simulink library "Linkage"  (R2025b)
settings: Solver=VariableStepAuto  StartTime=0.0  StopTime=10.0  RelTol=1e-3
undefined symbols (not defined in the file): Axle1D, AxleIn, Chassis, Init, RaceFix, RaceSpin, Vehicle, Visual, X, Y, Z
libraries: sm_lib x940, nesl_utility x136, fl_lib x6, Linkage_Systems x2, SteeringWheel x2, Linkage_Decoupled x2, AntiRollBar_Systems x1, Steer_Rack_None x1, Steer_Rack_WheelDrivenRack1UJoint x1
(part 1 of 25)
settings Model: Creator=andrei  LastModifiedBy=andrei

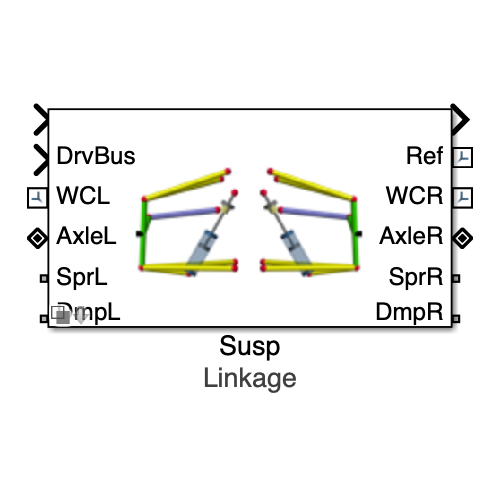
[thumbnail: Simulink's stored preview of the top-level diagram]
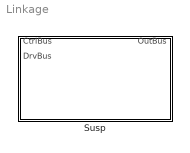
== system Linkage ==
  Susp : Subsystem  Variant=on  VariantControlMode=label  VariantControl=Variant1  LabelModeActiveChoice=Linkage  mask(Suspension and Steering){Susp=Chassis.SuspA1, Init=Init.Axle1, VariantLabel=Chassis.SuspA1.class.Value}
      mask prompts: Susp "Suspension Parameters"; Init "Initial Values"; VariantLabel "Variant Label"
      mask help: Models suspension and optional steering system for one axle. Option is chosen by string provided in Variant Label. The parameters for the selected option are contained in Suspension Parameters data structure.
      mask init:
      | curblk = gcb;
      | 
      | % Set variant for this block 
      | set_param(curblk,'LabelModeActiveChoice',VariantLabel);
      settings: AttributesFormatString=%<LabelModeActiveChoice>

== system Linkage/Susp ==
  "CtrlBus " : Inport
  DrvBus : Inport  Port=2
  Linkage : Subsystem  VariantControl=Linkage  mask(Linkage Suspension){}
      mask help: Models suspension using linkages, including double-wishbone and multi-link suspensions. This subsystem models the suspension, spring and damper parts, and optional steering system. The displacement of the springs and dampers are modeled here and the forces are modeled in a separate subsystem.
      mask Display: image('sm_car_vehicle_susp_linkage_IMAGE.png');
  Linkage Decoupled : Subsystem  VariantControl=Decoupled  mask(Linkage Decoupled){}
      mask help: Models suspension using a linkage where the stiffness and damping for the roll and heave degrees of freedom are decoupled. Includes suspension, spring and damper parts, and optional steering system. The displacement of the springs and dampers are modeled here and the forces are modeled in a separate subsystem.
      mask Display: image('sm_car_vehicle_susp_linkage_decouple_IMAGE.png');
  WCL : PMIOPort  Side=Left
  Ref : PMIOPort  Port=2  Side=Right
  WCR : PMIOPort  Port=3  Side=Right
  AxleL : PMIOPort  Port=4  Side=Left
  AxleR : PMIOPort  Port=5  Side=Right
  SprL : PMIOPort  Port=6  Side=Left
  SprR : PMIOPort  Port=7  Side=Right
  DmpL : PMIOPort  Port=8  Side=Left
  DmpR : PMIOPort  Port=9  Side=Right
  OutBus : Outport  VectorParamsAs1DForOutWhenUnconnected=off

== system Linkage/Susp/Linkage ==
  In Bus Element : Inport  PortName=CtrlBus  Element=Steer
  DrvBus : Inport  Port=2
  Anti Roll Bar : AntiRollBar_Systems/Anti Roll Bar  LabelModeActiveChoice=DroplinkRod  AntiRollBar=Susp.AntiRollBar  VariantLabel=Susp.AntiRollBar.class.Value
      settings: AttributesFormatString=%<LabelModeActiveChoice>
  Linkage L : Linkage_Systems/Linkage  VariantControl=Variant1  LabelModeActiveChoice=DoubleWishbone Pushrod  popup_leftRight=Left  Linkage=Susp.Linkage  InitLinkage=Init  VariantLabel=Susp.Linkage.class.Value
      settings: AttributesFormatString=%<ActiveVariant>
  Linkage R : Linkage_Systems/Linkage  VariantControl=Variant1  LabelModeActiveChoice=DoubleWishbone Pushrod  popup_leftRight=Right  Linkage=Susp.Linkage  InitLinkage=Init  VariantLabel=Susp.Linkage.class.Value
      settings: AttributesFormatString=%<ActiveVariant>
  Simscape Bus L : SimscapeBus  HierarchyStrings=RaceSpin;RaceFix;Axle1D;AxleIn
  Simscape Bus L1 : SimscapeBus  HierarchyStrings=RaceSpin;RaceFix;Axle1D;AxleIn
  Steer : Subsystem  Variant=on  VariantControlMode=label  VariantControl=Steer  LabelModeActiveChoice=RackWheel  mask{Steer=Susp.Steer, VariantLabel=Susp.Steer.class.Value}
      mask prompts: Steer "Steer Parameters"; VariantLabel "Variant Label"
      mask init:
      | curblk = gcb;
      | 
      | % Set variant for this block 
      | set_param(curblk,'LabelModeActiveChoice',VariantLabel);
      settings: AttributesFormatString=%<ActiveVariant>
      mask Display: disp(' ');
  Wheel Meas Left : Subsystem  mask(Wheel Measurements){popup_leftRight=Left}
      mask prompts: popup_leftRight "Left/Right"
      mask help: Calculates toe and camber angles based on orientation of wheel spin axis. To estimate steering axis inclination, the same measurements are done along the longitudinal axis (X) of the tire. Set Left/Right so that the sign of the logged toe and camber angles is associated with towards/away from vehicle center.
      mask init:
      | if(popup_leftRight == 1)
      |     rhs_tc = 1;
      | elseif(popup_leftRight == 2)
      |     rhs_tc = -1;
      | end
      mask TypeOptions popup_leftRight: Left | Right
  Wheel Meas Right : Subsystem  mask(Wheel Measurements){popup_leftRight=Right}
      mask prompts: popup_leftRight "Left/Right"
      mask help: Calculates toe and camber angles based on orientation of wheel spin axis. To estimate steering axis inclination, the same measurements are done along the longitudinal axis (X) of the tire. Set Left/Right so that the sign of the logged toe and camber angles is associated with towards/away from vehicle center.
      mask init:
      | if(popup_leftRight == 1)
      |     rhs_tc = 1;
      | elseif(popup_leftRight == 2)
      |     rhs_tc = -1;
      | end
      mask TypeOptions popup_leftRight: Left | Right
  WCL : PMIOPort  Side=Left
  Ref : PMIOPort  Port=2  Side=Right
  WCR : PMIOPort  Port=3  Side=Right
  AxleL : PMIOPort  Port=4  Side=Left
  AxleR : PMIOPort  Port=5  Side=Right
  SprL : PMIOPort  Port=6  Side=Left
  SprR : PMIOPort  Port=7  Side=Right
  DmpL : PMIOPort  Port=8  Side=Left
  DmpR : PMIOPort  Port=9  Side=Right
  Out Bus Element : Outport  VectorParamsAs1DForOutWhenUnconnected=off  PortName=OutBus  Element=Steer
  Out Bus Element1 : Outport  VectorParamsAs1DForOutWhenUnconnected=off  PortName=OutBus  Element=AntiRollBar
  Out Bus Element2 : Outport  VectorParamsAs1DForOutWhenUnconnected=off  PortName=OutBus  Element=WhlL
  Out Bus Element3 : Outport  VectorParamsAs1DForOutWhenUnconnected=off  PortName=OutBus  Element=WhlR
  Out Bus Element4 : Outport  VectorParamsAs1DForOutWhenUnconnected=off  PortName=OutBus  Element=LinkageR
  Out Bus Element5 : Outport  VectorParamsAs1DForOutWhenUnconnected=off  PortName=OutBus  Element=LinkageL
  wires:
  Wheel Meas Right/1(meas) -> Out Bus Element3/1
  Wheel Meas Left/1(meas) -> Out Bus Element2/1
  Anti Roll Bar/1 -> Out Bus Element1/1
  In Bus Element/1 -> Steer/2(CtrlBus)
  Steer/1(" meas") -> Out Bus Element/1
  DrvBus/1 -> Steer/1(DrvBus)
  Linkage R/1 -> Out Bus Element4/1
  Linkage L/1 -> Out Bus Element5/1
  connections:
  Linkage L/LConn8 -- Anti Roll Bar/LConn1
  Linkage R/LConn8 -- Anti Roll Bar/LConn3
  Linkage R/LConn5 -- Simscape Bus L1/LConn4
  Linkage L/LConn6 -- SprL/RConn1
  Simscape Bus L1/RConn1 -- AxleR/RConn1
  Linkage R/LConn4 -- Simscape Bus L1/LConn3
  Linkage R/LConn3 -- Simscape Bus L1/LConn2
  Linkage R/LConn2 -- Simscape Bus L1/LConn1
  Linkage R/LConn6 -- SprR/RConn1
  Linkage R/LConn7 -- DmpR/RConn1
  AxleL/RConn1 -- Simscape Bus L/RConn1
  Linkage L/LConn4 -- Simscape Bus L/LConn3
  Linkage L/LConn3 -- Simscape Bus L/LConn2
  Linkage L/LConn2 -- Simscape Bus L/LConn1
  Linkage L/LConn5 -- Simscape Bus L/LConn4
  Linkage L/LConn7 -- DmpL/RConn1
  Linkage L/RConn1 -- Steer/RConn1
  Wheel Meas Right/LConn2 -- Linkage R/LConn1 -- WCR/RConn1
  Wheel Meas Left/LConn2 -- Linkage L/LConn1 -- WCL/RConn1
  Wheel Meas Left/LConn1 -- Wheel Meas Right/LConn1 -- Steer/RConn2 -- Linkage R/RConn2 -- Linkage L/RConn2 -- Anti Roll Bar/LConn2 -- Ref/RConn1
  Linkage R/RConn1 -- Steer/RConn3

== system Linkage/Susp/Linkage Decoupled ==
  In Bus Element : Inport  PortName=CtrlBus  Element=Steer
  DrvBus : Inport  Port=2
  Linkage L : Linkage_Decoupled/Linkage  VariantControl=Variant1  LabelModeActiveChoice=DWDecoupled  popup_leftRight=Left  Linkage=Susp.Linkage  InitLinkage=Init  VariantLabel=Susp.Linkage.class.Value
      settings: AttributesFormatString=%<ActiveVariant>
  Linkage R : Linkage_Decoupled/Linkage  VariantControl=Variant1  LabelModeActiveChoice=DWDecoupled  popup_leftRight=Right  Linkage=Susp.Linkage  InitLinkage=Init  VariantLabel=Susp.Linkage.class.Value
      settings: AttributesFormatString=%<ActiveVariant>
  RollHeave Decouple : Subsystem  VariantControl=Variant1  mask(Roll and Heave Spring Dampers){hp_pushrod=Susp.Linkage.Pushrod.sBellcrank.Value, hp_bcr_pivot=Susp.Linkage.Bellcrank.sPivot.Value, hp_bcr_shock_heaveL=Susp.Linkage.Shock.Heave.sLeft.Value, hp_bcr_shock_heaveR=Susp.Linkage.Shock.Heave.sRight.Value, hp_bcr_shock_rollL=Susp.Linkage.Shock.Roll.sLeft.Value, hp_bcr_shock_rollR=Susp.Linkage.Shock.Roll.sRight.Value, shock_pist_mass_heave=Susp.Linkage.Shock.Heave.mPiston.Value, shock_pist_mass_roll=Susp.Linkage.Shock.Roll.mPiston.Value, shock_cyl_mass_heave=Susp.Linkage.Shock.Heave.mCylinder.Value, shock_cyl_mass_roll=Susp.Linkage.Shock.Roll.mCylinder.Value, up_lim_bumpstop_heave=Susp.Linkage.Endstop.Heave.xMax.Value, up_lim_bumpstop_roll=Susp.Linkage.Endstop.Roll.xMax.Value, low_lim_bumpstop_heave=Susp.Linkage.Endstop.Heave.xMin.Value, low_lim_bumpstop_roll=Susp.Linkage.Endstop.Roll.xMin.Value, clr_conn_shock=Visual.hp.clr, opc_conn_shock=Visual.hp.opc, size_conn_shock=Visual.hp.rad, clr_shock_cyl=Visual.Shock.cyl.clr, opc_shock_cyl=Visual.part.opc, radius_shock_cyl=Visual.Shock.cyl.rad, clr_shock_piston=Visual.Shock.piston.clr, opc_shock_piston=Visual.part.opc, clr_shock_bumpstop=Visual.Shock.bumpstop.clr, opc_shock_bumpstop=Visual.part.opc, deadvol_len_shock_cyl=Visual.Shock.dead_length, piston_len_shock=Visual.Shock.piston.len, cyl_cap_len_shock=Visual.Shock.cap.len, bumpstop_len_shock=Visual.Shock.bumpstop.len}
      mask prompts: hp_pushrod "HP Pushrod Inner  [xyz] (m)"; hp_bcr_pivot "HP Bellcrank Pivot [xyz] (m)"; deadvol_len_shock_cyl "Dead Volume Height (m)"; piston_len_shock "Piston Length (m)"; cyl_cap_len_shock "Cylinder Cap Length (m)"; bumpstop_len_shock "Bumpstop Length (m)"
      mask help: Models springs and dampers in a suspension design that decouples stiffness and damping for body roll and heave.
      mask init:
      | % Code to mirror hardpoint about vehicle xz plane
      | % and the plane defined by the bellcrank pivot axis
      | % and the y axis of the vehicle
      | % Code not used so that points can be specified independently
      | % Left here as a reference.
      | %{
      |  
      | a1 = atan2(hp_pushrod(1)-hp_bcr_pivot(1)   ,hp_pushrod(3)-hp_bcr_pivot(3));
      | a2 = atan2(hp_bcr_shock_roll(1)-hp_bcr_pivot(1),hp_bcr_shock_roll(3)-hp_bcr_pivot(3));
      | d_roll2piv = norm(hp_bcr_shock_roll([1 3])-hp_bcr_pivot([1 3]));
      | d_roll_mirror_axis = d_roll2piv*cos(a2-a1);
      | mirr_dx = d_roll_mirror_axis*sin(a1);
      | mirr_dz = d_roll_mirror_axis*cos(a1);
      | hp_bcr_shock_roll_r = ...
      |     [hp_bcr_shock_roll(1)-2*mirr_dx -hp_bcr_shock_roll(2) hp_bcr_shock_roll(3)-2*mirr_dz]
      | %}
      mask TypeOptions shock_pist_mass_heave: Shock Heave/shock_pist_mass
      mask TypeOptions shock_pist_mass_roll: Shock Roll/shock_pist_mass
      mask TypeOptions shock_cyl_mass_heave: Shock Heave/shock_cyl_mass
      mask TypeOptions shock_cyl_mass_roll: Shock Roll/shock_cyl_mass
      mask TypeOptions up_lim_bumpstop_heave: Shock Heave/up_lim_bumpstop
      mask TypeOptions up_lim_bumpstop_roll: Shock Roll/up_lim_bumpstop
      mask TypeOptions low_lim_bumpstop_heave: Shock Heave/low_lim_bumpstop
      mask TypeOptions low_lim_bumpstop_roll: Shock Roll/low_lim_bumpstop
      mask TypeOptions clr_conn_shock: Shock Heave/clr_conn_shock | Shock Roll/clr_conn_shock
      mask TypeOptions opc_conn_shock: Shock Heave/opc_conn_shock | Shock Roll/opc_conn_shock
      mask TypeOptions size_conn_shock: Shock Heave/size_conn_shock | Shock Roll/size_conn_shock
      mask TypeOptions clr_shock_cyl: Shock Heave/clr_shock_cyl | Shock Roll/clr_shock_cyl
      mask TypeOptions opc_shock_cyl: Shock Heave/opc_shock_cyl | Shock Roll/opc_shock_cyl
      mask TypeOptions radius_shock_cyl: Shock Heave/radius_shock_cyl | Shock Roll/radius_shock_cyl
      mask TypeOptions clr_shock_piston: Shock Heave/clr_shock_piston | Shock Roll/clr_shock_piston
      mask TypeOptions opc_shock_piston: Shock Heave/opc_shock_piston | Shock Roll/opc_shock_piston
      mask TypeOptions clr_shock_bumpstop: Shock Heave/clr_shock_bumpstop | Shock Roll/clr_shock_bumpstop
      mask TypeOptions opc_shock_bumpstop: Shock Heave/opc_shock_bumpstop | Shock Roll/opc_shock_bumpstop
      mask TypeOptions deadvol_len_shock_cyl: Shock Heave/deadvol_len_shock_cyl | Shock Roll/deadvol_len_shock_cyl
      mask TypeOptions piston_len_shock: Shock Heave/piston_len_shock | Shock Roll/piston_len_shock
      mask TypeOptions cyl_cap_len_shock: Shock Heave/cyl_cap_len_shock | Shock Roll/cyl_cap_len_shock
      mask TypeOptions bumpstop_len_shock: Shock Heave/bumpstop_len_shock | Shock Roll/bumpstop_len_shock
      mask DialogControl cont_hp Prompt: Hardpoints
      mask DialogControl text_hp_left Prompt: Left
      mask DialogControl text_hp_right Prompt: Right
      mask DialogControl text_hp_heave Prompt: Heave [xyz] (m)
      mask DialogControl text_hp_roll Prompt: Roll [xyz] (m)
      mask DialogControl cont_shock Prompt: Shock
      mask DialogControl text_shock_parts_blank Prompt: Parts
      mask DialogControl text_shock_heave Prompt: Heave
      mask DialogControl text_shock_roll Prompt: Roll
      mask DialogControl text_shock_pistm Prompt: Piston Mass (kg)
      mask DialogControl text_shock_cylm Prompt: Cylinder Mass (kg)
      mask DialogControl text_shock_bumpstop_par Prompt: Bumpstop
      mask DialogControl text_bump_ul Prompt: Upper Limit (m)
      mask DialogControl text_bump_low Prompt: Lower Limit (m)
      mask DialogControl cont_vis_shock Prompt: Visualization
      mask DialogControl text_clr_shock Prompt: Color  [RGB]
      mask DialogControl text_opc_shock Prompt: Opac. (0-1)
      mask DialogControl text_size_shock Prompt: Size (m)
      mask DialogControl text_conn_shock Prompt: Connections
      mask DialogControl text_shock_shock Prompt: Cylinder
      mask DialogControl text_shock_piston Prompt: Piston
      mask DialogControl text_piston_radius Prompt: <cylinder radius>
      mask DialogControl text_shock_bumpstop Prompt: Bumpstop
      mask DialogControl text_bumpstop_radius Prompt: <cylinder radius>
      mask Display: image('sm_car_vehicle_linkage_rollHeaveDecouple_IMAGE.png');
  Simscape Bus L : SimscapeBus  HierarchyStrings=RaceSpin;RaceFix;Axle1D;AxleIn
  Simscape Bus L1 : SimscapeBus  HierarchyStrings=RaceSpin;RaceFix;Axle1D;AxleIn
  Steer : Subsystem  Variant=on  VariantControlMode=label  VariantControl=Steer  LabelModeActiveChoice=WheelDrivenRack1UJoint  mask{Steer=Susp.Steer, VariantLabel=Susp.Steer.class.Value}
      mask prompts: Steer "Steer Parameters"; VariantLabel "Variant Label"
      mask init:
      | curblk = gcb;
      | 
      | % Set variant for this block 
      | set_param(curblk,'LabelModeActiveChoice',VariantLabel);
      settings: AttributesFormatString=%<ActiveVariant>
      mask Display: disp(' ');
  Wheel Meas Left : Subsystem  mask(Wheel Measurements){popup_leftRight=Left}
      mask prompts: popup_leftRight "Left/Right"
      mask help: Calculates toe and camber angles based on orientation of wheel spin axis. To estimate steering axis inclination, the same measurements are done along the longitudinal axis (X) of the tire. Set Left/Right so that the sign of the logged toe and camber angles is associated with towards/away from vehicle center.
      mask init:
      | if(popup_leftRight == 1)
      |     rhs_tc = 1;
      | elseif(popup_leftRight == 2)
      |     rhs_tc = -1;
      | end
      mask TypeOptions popup_leftRight: Left | Right
  Wheel Meas Right : Subsystem  mask(Wheel Measurements){popup_leftRight=Right}
      mask prompts: popup_leftRight "Left/Right"
      mask help: Calculates toe and camber angles based on orientation of wheel spin axis. To estimate steering axis inclination, the same measurements are done along the longitudinal axis (X) of the tire. Set Left/Right so that the sign of the logged toe and camber angles is associated with towards/away from vehicle center.
      mask init:
      | if(popup_leftRight == 1)
      |     rhs_tc = 1;
      | elseif(popup_leftRight == 2)
      |     rhs_tc = -1;
      | end
      mask TypeOptions popup_leftRight: Left | Right
  WCL : PMIOPort  Side=Left
  Ref : PMIOPort  Port=2  Side=Right
  WCR : PMIOPort  Port=3  Side=Right
  AxleL : PMIOPort  Port=4  Side=Left
  AxleR : PMIOPort  Port=5  Side=Right
  SprL : PMIOPort  Port=6  Side=Left
  SprR : PMIOPort  Port=7  Side=Right
  DmpL : PMIOPort  Port=8  Side=Left
  DmpR : PMIOPort  Port=9  Side=Right
  Out Bus Element : Outport  VectorParamsAs1DForOutWhenUnconnected=off  PortName=OutBus  Element=Steer
  Out Bus Element1 : Outport  VectorParamsAs1DForOutWhenUnconnected=off  PortName=OutBus  Element=RollHeave
  Out Bus Element2 : Outport  VectorParamsAs1DForOutWhenUnconnected=off  PortName=OutBus  Element=WhlL
  Out Bus Element3 : Outport  VectorParamsAs1DForOutWhenUnconnected=off  PortName=OutBus  Element=WhlR
  Out Bus Element4 : Outport  VectorParamsAs1DForOutWhenUnconnected=off  PortName=OutBus  Element=LinkageR
  Out Bus Element5 : Outport  VectorParamsAs1DForOutWhenUnconnected=off  PortName=OutBus  Element=LinkageL
  wires:
  Wheel Meas Right/1(meas) -> Out Bus Element3/1
  Wheel Meas Left/1(meas) -> Out Bus Element2/1
  In Bus Element/1 -> Steer/2(CtrlBus)
  Steer/1(" meas") -> Out Bus Element/1
  DrvBus/1 -> Steer/1(DrvBus)
  RollHeave Decouple/1(meas) -> Out Bus Element1/1
  Linkage R/1 -> Out Bus Element4/1
  Linkage L/1 -> Out Bus Element5/1
  connections:
  RollHeave Decouple/LConn1 -- Linkage L/LConn6
  Linkage R/LConn5 -- Simscape Bus L1/LConn4
  Simscape Bus L1/RConn1 -- AxleR/RConn1
  Linkage R/LConn4 -- Simscape Bus L1/LConn3
  Linkage R/LConn3 -- Simscape Bus L1/LConn2
  Linkage R/LConn2 -- Simscape Bus L1/LConn1
  AxleL/RConn1 -- Simscape Bus L/RConn1
  Linkage L/LConn4 -- Simscape Bus L/LConn3
  Linkage L/LConn3 -- Simscape Bus L/LConn2
  Linkage L/LConn2 -- Simscape Bus L/LConn1
  Linkage L/LConn5 -- Simscape Bus L/LConn4
  Steer/RConn1 -- Linkage L/RConn1
  Wheel Meas Right/LConn2 -- Linkage R/LConn1 -- WCR/RConn1
  Wheel Meas Left/LConn2 -- Linkage L/LConn1 -- WCL/RConn1
  Steer/RConn2 -- Wheel Meas Right/LConn1 -- Wheel Meas Left/LConn1 -- Linkage R/RConn2 -- Ref/RConn1 -- Linkage L/RConn2
  Steer/RConn3 -- Linkage R/RConn1
  RollHeave Decouple/LConn2 -- Linkage L/LConn7
  RollHeave Decouple/LConn7 -- Linkage R/LConn7
  RollHeave Decouple/LConn8 -- Linkage R/LConn6
  DmpL/RConn1 -- RollHeave Decouple/LConn4
  SprL/RConn1 -- RollHeave Decouple/LConn3
  DmpR/RConn1 -- RollHeave Decouple/LConn6
  SprR/RConn1 -- RollHeave Decouple/LConn5

== system Linkage/Susp/Linkage/Steer ==
  DrvBus : Inport
  CtrlBus : Inport  Port=2
  None : Steer_Rack_None/None  SystemSampleTime=-1  VariantControl=None  VariantActivationTime=update diagram  EmptyChoice=off  PassThrough=off  PassThroughVariantControl=(default)  EmptyChoiceVariantControl=(default)  AllowFlexibleInterface=on  Latency=0  AutoFrameSizeCalculation=off
  Rack Wheel : Subsystem  Tag=PublishSubsystem  AncestorBlock=Steer_Rack_Wheel/Rack Wheel  VariantControl=RackWheel  mask(Steering System with Rack Actuation){hp_wheel=Vehicle.Chassis.SuspA1.Steer.Wheel.sMount.Value, wheel_axis_incl=Vehicle.Chassis.SuspA1.Steer.Wheel.aAxis.Value, hp_mt_rack=Vehicle.Chassis.SuspA1.Steer.Rack.sMount.Value, hp_out_rack=Vehicle.Chassis.SuspA1.Steer.Rack.sOutboard.Value, Wheel=Steer.Wheel, rack_mass=Vehicle.Chassis.SuspA1.Steer.Rack.m.Value, whl2rack_whlangle=Vehicle.Chassis.SuspA1.Steer.Ratio_Table.aWheel.Value, whl2rack_rackdisp=Vehicle.Chassis.SuspA1.Steer.Ratio_Table.xRack.Value, whl2rack_filter=1/Vehicle.Chassis.SuspA1.Steer.Rack.fActuatorCutoff.Value, clr_rack=Visual.SteeringRack.clr, opc_rack=Visual.part.opc, radius_rack=Visual.SteeringRack.rad, clr_connhp=Visual.hp.clr, opc_connhp=Visual.hp.opc, size_connhp=Visual.hp.rad, clr_wheel=Visual.SteeringWheel.clr, opc_wheel=Visual.part.opc, DriverHuman=Steer.DriverHuman}
      mask prompts: hp_wheel "HP Wheel [xyz] (m)"; wheel_axis_incl "Wheel Axis Angle (rad)"; hp_mt_rack "HP Rack Mount [xyz] (m)"; hp_out_rack "HP Track Rod Inboard [xyz] (m)"; whl2rack_whlangle "Wheel Angle (deg)"; whl2rack_rackdisp "Rack Travel (m)"; whl2rack_filter "Rack Motion Filter (sec)"; DriverHuman "Driver Human (structure)"
      mask help: Steering wheel angle converted to rack displacement by lookup table. Steering wheel is present and rotates to match rack displacement (visualization only). Shafts are not present.
      mask TypeOptions hp_wheel:
      | Ref to Wheel/Transform
      | HP Wheel/TranslationCartesianOffset
      mask TypeOptions hp_mt_rack:
      | Ref to Rack/Transform
      | HP Rack/TranslationCartesianOffset
      mask TypeOptions hp_out_rack: Rack/hp_out
      mask TypeOptions rack_mass: Rack/rack_mass
      mask TypeOptions whl2rack_whlangle:
      | Wheel Angle to
      | Rack Displacement/BreakpointsForDimension1
      mask TypeOptions whl2rack_rackdisp:
      | Wheel Angle to
      | Rack Displacement/Table
      mask TypeOptions whl2rack_filter: Physical Signal/InputFilterTimeConstant
      mask TypeOptions clr_rack: Rack/clr_rack
      mask TypeOptions opc_rack: Rack/opc_rack
      mask TypeOptions radius_rack: Rack/radius_rack
      mask TypeOptions clr_connhp:
      | Ref to Rack/Vis
      | Rack
      | Housing/GraphicDiffuseColor
      mask TypeOptions opc_connhp:
      | Ref to Rack/Vis
      | Rack
      | Housing/GraphicOpacity
      mask TypeOptions size_connhp:
      | Ref to Rack/Vis
      | Rack
      | Housing/SphereRadius
      mask TypeOptions clr_wheel: Wheel/clr_wheel
      mask TypeOptions opc_wheel: Wheel/opc_wheel
      mask DialogControl cont_steer Prompt: Steer
      mask DialogControl grp_strparts Prompt: Parts
      mask DialogControl text_strparts_len Prompt: Length/Radius (m)
      mask DialogControl text_strparts_mass Prompt: Mass (kg)
      mask DialogControl text_strparts_wheel Prompt: Wheel
      mask DialogControl text_strparts_wheel_m Prompt: <CAD file>
      mask DialogControl text_strparts_rack Prompt: Rack
      mask DialogControl text_strparts_rack_len Prompt: <HP Rod Inboard>
      mask DialogControl grp_whl2rack Prompt: Wheel to Rack
      mask DialogControl cont_vis_steer Prompt: Visualization
      mask DialogControl text_steer_vis_clr Prompt: Color [RGB]
      mask DialogControl text_steer_vis_opc Prompt: Opac. (0-1)
      mask DialogControl text_steer_vis_size Prompt: Size (m)
      mask DialogControl text_steer_vis_rack Prompt: Rack
      mask DialogControl text_steer_vis_connhp Prompt: Connections, HP
      mask DialogControl text_steer_vis_wheel Prompt: Wheel
      mask DialogControl text_wheel_size Prompt: <CAD File>
      mask DialogControl cont_driver_human Prompt: Driver Human
  Wheel Driven Rack 1UJoint : Steer_Rack_WheelDrivenRack1UJoint/Wheel Driven Rack 1UJoint  Tag=PublishSubsystem  VariantControl=WheelDrivenRack1UJoint  hp_wheel=Vehicle.Chassis.SuspA1.Steer.Wheel.sMount.Value  wheel_axis_incl=Vehicle.Chassis.SuspA1.Steer.Wheel.aAxis.Value  hp_mt_rack=Vehicle.Chassis.SuspA1.Steer.Rack.sMount.Value  hp_out_rack=Vehicle.Chassis.SuspA1.Steer.Rack.sOutboard.Value  hp_pinion=Vehicle.Chassis.SuspA1.Steer.Pinion.sMount.Value  Wheel=Steer.Wheel  len_sha_u=Vehicle.Chassis.SuspA1.Steer.Shaft_Upper.xLength.Value  sha_u_mass=Steer.Shaft_Upper.m.Value  sha_l_mass=Steer.Shaft_Lower.m.Value  rad_pinion=Vehicle.Chassis.SuspA1.Steer.Pinion.xRad.Value  pinion_mass=Steer.Pinion.m.Value  rack_mass=Steer.Rack.m.Value  whl2steer_filter=1/Vehicle.Chassis.SuspA1.Steer.Rack.fActuatorCutoff.Value  clr_rack=Visual.SteeringRack.clr  opc_rack=Visual.part.opc  radius_rack=Visual.SteeringRack.rad  clr_shaft=Visual.SteeringShafts.clr  opc_shaft=Visual.part.opc  size_shaft=Visual.SteeringShafts.rad  clr_pinion=Visual.SteeringPinion.clr  opc_pinion=Visual.part.opc  len_pinion=Visual.SteeringPinion.len  clr_connhp=Visual.hp.clr  opc_connhp=Visual.hp.opc  size_connhp=Visual.hp.rad  clr_wheel=Visual.SteeringWheel.clr  opc_wheel=Visual.part.opc  DriverHuman=Steer.DriverHuman
  Wheel Driven Rack 1UJoint1 : Subsystem  Tag=PublishSubsystem  VariantControl=WheelDrivenRack1UJoint1  mask(Steering System with Wheel Actuation){hp_wheel=Steer.Wheel.sMount.Value, wheel_axis_incl=Steer.Wheel.aAxis.Value, hp_mt_rack=Steer.Rack.sMount.Value, hp_out_rack=Steer.Rack.sOutboard.Value, hp_pinion=Steer.Pinion.sMount.Value, Wheel=Steer.Wheel, len_sha_u=Steer.Shaft_Upper.xLength.Value, sha_u_mass=Steer.Shaft_Upper.m.Value, sha_l_mass=Steer.Shaft_Lower.m.Value, rad_pinion=Steer.Pinion.xRad.Value, pinion_mass=Steer.Pinion.m.Value, rack_mass=Steer.Rack.m.Value, whl2steer_filter=1/Steer.Rack.fActuatorCutoff.Value, clr_rack=Visual.SteeringRack.clr, opc_rack=Visual.part.opc, radius_rack=Visual.SteeringRack.rad, clr_shaft=Visual.SteeringShafts.clr, opc_shaft=Visual.part.opc, size_shaft=Visual.SteeringShafts.rad, clr_pinion=Visual.SteeringPinion.clr, opc_pinion=Visual.part.opc, len_pinion=Visual.SteeringPinion.len, clr_connhp=Visual.hp.clr, opc_connhp=Visual.hp.opc, size_connhp=Visual.hp.rad, clr_wheel=Visual.SteeringWheel.clr, opc_wheel=Visual.part.opc, DriverHuman=Steer.DriverHuman}
      mask prompts: hp_wheel "HP Wheel [xyz] (m)"; wheel_axis_incl "Wheel Axis Angle (rad)"; hp_mt_rack "HP Rack Mount [xyz] (m)"; hp_out_rack "HP Track Rod Inboard [xyz] (m)"; hp_pinion "HP Pinion [xyz] (m)"; whl2steer_filter "Steer Motion Filter (sec)"; DriverHuman "Driver Human (structure)"
      mask help: Actuation is applied to steering wheel and transmitted to rack via shafts in steering column. Assumes constant gear ratio between pinion and rack.
      mask init:
      | % Calculate inclination of pinion gear about rack travel axis
      | pinion_incl = atan2(hp_mt_rack(1)-hp_pinion(1),hp_mt_rack(3)-hp_pinion(3));
      | 
      | % Calculate location of universal joint
      | hp_col_upper = hp_wheel  + [+len_sha_u*cos(wheel_axis_incl)  0 -len_sha_u*sin(wheel_axis_incl)];
      mask TypeOptions hp_wheel:
      | Ref to Wheel/Transform
      | HP Wheel/TranslationCartesianOffset
      mask TypeOptions hp_mt_rack:
      | Ref to Rack/Transform
      | HP Rack/TranslationCartesianOffset
      mask TypeOptions hp_out_rack: Rack/hp_out
      mask TypeOptions rack_mass: Rack/rack_mass
      mask TypeOptions whl2steer_filter: Physical Signal/InputFilterTimeConstant
      mask TypeOptions clr_rack: Rack/clr_rack
      mask TypeOptions opc_rack: Rack/opc_rack
      mask TypeOptions radius_rack: Rack/radius_rack
      mask TypeOptions clr_shaft:
      | Shaft
      | Steering/Shaft/GraphicDiffuseColor | Shaft
      | Lower/Shaft/GraphicDiffuseColor | Shaft
      | Intermediate/Shaft/GraphicDiffuseColor
      mask TypeOptions opc_shaft:
      | Shaft
      | Steering/Shaft/GraphicOpacity | Shaft
      | Lower/Shaft/GraphicOpacity | Shaft
      | Intermediate/Shaft/GraphicOpacity
      mask TypeOptions size_shaft:
      | Shaft
      | Steering/Shaft/CylinderRadius | Shaft
      | Lower/Shaft/CylinderRadius | Shaft
      | Intermediate/Shaft/CylinderRadius
      mask TypeOptions clr_pinion: Pinion/Pinion/GraphicDiffuseColor
      mask TypeOptions opc_pinion: Pinion/Pinion/GraphicOpacity
      mask TypeOptions len_pinion: Pinion/Pinion/CylinderLength
      mask TypeOptions clr_connhp:
      | Ref to Rack/Vis
      | Rack
      | Housing/GraphicDiffuseColor | HPs/HP Lower Col/GraphicDiffuseColor | HPs/HP Pinion/GraphicDiffuseColor | HPs/HP Upper Col/GraphicDiffuseColor
      mask TypeOptions opc_connhp:
      | Ref to Rack/Vis
      | Rack
      | Housing/GraphicOpacity | HPs/HP Lower Col/GraphicOpacity | HPs/HP Pinion/GraphicOpacity | HPs/HP Upper Col/GraphicOpacity
      mask TypeOptions size_connhp:
      | Ref to Rack/Vis
      | Rack
      | Housing/SphereRadius | HPs/HP Lower Col/SphereRadius | HPs/HP Pinion/SphereRadius | HPs/HP Upper Col/SphereRadius
      mask TypeOptions clr_wheel: Wheel/clr_wheel
      mask TypeOptions opc_wheel: Wheel/opc_wheel
      mask DialogControl cont_steer Prompt: Steer
      mask DialogControl grp_strparts Prompt: Parts
      mask DialogControl text_strparts_len Prompt: Length/Radius (m)
      mask DialogControl text_strparts_mass Prompt: Mass (kg)
      mask DialogControl text_strparts_wheel Prompt: Wheel
      mask DialogControl text_strparts_wheel_m Prompt: <CAD file>
      mask DialogControl text_strparts_sha_u Prompt: Upper Shaft
      mask DialogControl text_strparts_sha_i Prompt: Lower Shaft
      mask DialogControl text_strparts_sha_i_len Prompt: <length upper, lower>
      mask DialogControl text_strparts_pinion Prompt: Pinion
      mask DialogControl text_strparts_rack Prompt: Rack
      mask DialogControl text_strparts_rack_len Prompt: <HP Rod Inboard>
      mask DialogControl grp_steering Prompt: Steering Input
      mask DialogControl cont_vis_steer Prompt: Visualization
      mask DialogControl text_steer_vis_clr Prompt: Color [RGB]
      mask DialogControl text_steer_vis_opc Prompt: Opac. (0-1)
      mask DialogControl text_steer_vis_size Prompt: Size (m)
      mask DialogControl text_steer_vis_rack Prompt: Rack
      mask DialogControl text_steer_vis_shafts Prompt: Shafts
      mask DialogControl text_steer_vis_pinion Prompt: Pinion
      mask DialogControl text_steer_vis_connhp Prompt: Connections, HP
      mask DialogControl text_steer_vis_wheel Prompt: Wheel
      mask DialogControl text_steer_size_wheel Prompt: <CAD File>
      mask DialogControl cont_driver_human Prompt: Driver Human
  Wheel Driven Rack 1UJoint2 : Subsystem  Tag=PublishSubsystem  VariantControl=WheelDrivenRack1UJoint2  mask(Steering System with Wheel Actuation){hp_wheel=Steer.Wheel.sMount.Value, wheel_axis_incl=Steer.Wheel.aAxis.Value, hp_mt_rack=Steer.Rack.sMount.Value, hp_out_rack=Steer.Rack.sOutboard.Value, hp_pinion=Steer.Pinion.sMount.Value, Wheel=Steer.Wheel, len_sha_u=Steer.Shaft_Upper.xLength.Value, sha_u_mass=Steer.Shaft_Upper.m.Value, sha_l_mass=Steer.Shaft_Lower.m.Value, rad_pinion=Steer.Pinion.xRad.Value, pinion_mass=Steer.Pinion.m.Value, rack_mass=Steer.Rack.m.Value, whl2steer_filter=1/Steer.Rack.fActuatorCutoff.Value, clr_rack=Visual.SteeringRack.clr, opc_rack=Visual.part.opc, radius_rack=Visual.SteeringRack.rad, clr_shaft=Visual.SteeringShafts.clr, opc_shaft=Visual.part.opc, size_shaft=Visual.SteeringShafts.rad, clr_pinion=Visual.SteeringPinion.clr, opc_pinion=Visual.part.opc, len_pinion=Visual.SteeringPinion.len, clr_connhp=Visual.hp.clr, opc_connhp=Visual.hp.opc, size_connhp=Visual.hp.rad, clr_wheel=Visual.SteeringWheel.clr, opc_wheel=Visual.part.opc, DriverHuman=Steer.DriverHuman}
      mask prompts: hp_wheel "HP Wheel [xyz] (m)"; wheel_axis_incl "Wheel Axis Angle (rad)"; hp_mt_rack "HP Rack Mount [xyz] (m)"; hp_out_rack "HP Track Rod Inboard [xyz] (m)"; hp_pinion "HP Pinion [xyz] (m)"; whl2steer_filter "Steer Motion Filter (sec)"; DriverHuman "Driver Human (structure)"
      mask help: Actuation is applied to steering wheel and transmitted to rack via shafts in steering column. Assumes constant gear ratio between pinion and rack.
      mask init: same as Linkage/Susp/Linkage/Steer/Wheel Driven Rack 1UJoint1
      mask TypeOptions hp_wheel:
      | Ref to Wheel/Transform
      | HP Wheel/TranslationCartesianOffset
      mask TypeOptions hp_mt_rack:
      | Ref to Rack/Transform
      | HP Rack/TranslationCartesianOffset
      mask TypeOptions hp_out_rack: Rack/hp_out
      mask TypeOptions rack_mass: Rack/rack_mass
      mask TypeOptions whl2steer_filter: Physical Signal/InputFilterTimeConstant
      mask TypeOptions clr_rack: Rack/clr_rack
      mask TypeOptions opc_rack: Rack/opc_rack
      mask TypeOptions radius_rack: Rack/radius_rack
      mask TypeOptions clr_shaft:
      | Shaft
      | Steering/Shaft/GraphicDiffuseColor | Shaft
      | Lower/Shaft/GraphicDiffuseColor | Shaft
      | Intermediate/Shaft/GraphicDiffuseColor
      mask TypeOptions opc_shaft:
      | Shaft
      | Steering/Shaft/GraphicOpacity | Shaft
      | Lower/Shaft/GraphicOpacity | Shaft
      | Intermediate/Shaft/GraphicOpacity
      mask TypeOptions size_shaft:
      | Shaft
      | Steering/Shaft/CylinderRadius | Shaft
      | Lower/Shaft/CylinderRadius | Shaft
      | Intermediate/Shaft/CylinderRadius
      mask TypeOptions clr_pinion: Pinion/Pinion/GraphicDiffuseColor
      mask TypeOptions opc_pinion: Pinion/Pinion/GraphicOpacity
      mask TypeOptions len_pinion: Pinion/Pinion/CylinderLength
      mask TypeOptions clr_connhp:
      | Ref to Rack/Vis
      | Rack
      | Housing/GraphicDiffuseColor | HPs/HP Lower Col/GraphicDiffuseColor | HPs/HP Pinion/GraphicDiffuseColor | HPs/HP Upper Col/GraphicDiffuseColor
      mask TypeOptions opc_connhp:
      | Ref to Rack/Vis
      | Rack
      | Housing/GraphicOpacity | HPs/HP Lower Col/GraphicOpacity | HPs/HP Pinion/GraphicOpacity | HPs/HP Upper Col/GraphicOpacity
      mask TypeOptions size_connhp:
      | Ref to Rack/Vis
      | Rack
      | Housing/SphereRadius | HPs/HP Lower Col/SphereRadius | HPs/HP Pinion/SphereRadius | HPs/HP Upper Col/SphereRadius
      mask TypeOptions clr_wheel: Wheel/clr_wheel
      mask TypeOptions opc_wheel: Wheel/opc_wheel
      mask DialogControl cont_steer Prompt: Steer
      mask DialogControl grp_strparts Prompt: Parts
      mask DialogControl text_strparts_len Prompt: Length/Radius (m)
      mask DialogControl text_strparts_mass Prompt: Mass (kg)
      mask DialogControl text_strparts_wheel Prompt: Wheel
      mask DialogControl text_strparts_wheel_m Prompt: <CAD file>
      mask DialogControl text_strparts_sha_u Prompt: Upper Shaft
      mask DialogControl text_strparts_sha_i Prompt: Lower Shaft
      mask DialogControl text_strparts_sha_i_len Prompt: <length upper, lower>
      mask DialogControl text_strparts_pinion Prompt: Pinion
      mask DialogControl text_strparts_rack Prompt: Rack
      mask DialogControl text_strparts_rack_len Prompt: <HP Rod Inboard>
      mask DialogControl grp_steering Prompt: Steering Input
      mask DialogControl cont_vis_steer Prompt: Visualization
      mask DialogControl text_steer_vis_clr Prompt: Color [RGB]
      mask DialogControl text_steer_vis_opc Prompt: Opac. (0-1)
      mask DialogControl text_steer_vis_size Prompt: Size (m)
      mask DialogControl text_steer_vis_rack Prompt: Rack
      mask DialogControl text_steer_vis_shafts Prompt: Shafts
      mask DialogControl text_steer_vis_pinion Prompt: Pinion
      mask DialogControl text_steer_vis_connhp Prompt: Connections, HP
      mask DialogControl text_steer_vis_wheel Prompt: Wheel
      mask DialogControl text_steer_size_wheel Prompt: <CAD File>
      mask DialogControl cont_driver_human Prompt: Driver Human
  Wheel Driven Rack 1UJoint3 : Subsystem  Tag=PublishSubsystem  AncestorBlock=|  VariantControl=WheelDrivenRack1UJoint3  mask(Steering System with Wheel Actuation){hp_wheel=Steer.Wheel.sMount.Value, wheel_axis_incl=Steer.Wheel.aAxis.Value, hp_mt_rack=Steer.Rack.sMount.Value, hp_out_rack=Steer.Rack.sOutboard.Value, Wheel=Steer.Wheel, len_sha_u=Steer.Shaft_Upper.xLength.Value, sha_u_mass=Steer.Shaft_Upper.m.Value, sha_l_mass=Steer.Shaft_Lower.m.Value, rad_pinion=Steer.Pinion.xRad.Value, pinion_mass=Steer.Pinion.m.Value, rack_mass=Steer.Rack.m.Value, whl2steer_filter=1/Steer.Rack.fActuatorCutoff.Value, clr_rack=Visual.SteeringRack.clr, opc_rack=Visual.part.opc, radius_rack=Visual.SteeringRack.rad, clr_shaft=Visual.SteeringShafts.clr, opc_shaft=Visual.part.opc, size_shaft=Visual.SteeringShafts.rad, clr_pinion=Visual.SteeringPinion.clr, opc_pinion=Visual.part.opc, len_pinion=Visual.SteeringPinion.len, clr_connhp=Visual.hp.clr, opc_connhp=Visual.hp.opc, size_connhp=Visual.hp.rad, clr_wheel=Visual.SteeringWheel.clr, opc_wheel=Visual.part.opc, DriverHuman=Steer.DriverHuman}
      | Steer_Rack_WheelDrivenRack1UJoint/Wheel
      | Driven
      | Rack
      | 1UJoint
      mask prompts: hp_wheel "HP Wheel [xyz] (m)"; wheel_axis_incl "Wheel Axis Angle (rad)"; hp_mt_rack "HP Rack Mount [xyz] (m)"; hp_out_rack "HP Track Rod Inboard [xyz] (m)"; whl2steer_filter "Steer Motion Filter (sec)"; DriverHuman "Driver Human (structure)"
      mask help: Actuation is applied to steering wheel and transmitted to rack via shafts in steering column. Assumes constant gear ratio between pinion and rack.
      mask init:
      | % Calculate the pinion inclination only based on pinion radius, wheel and
      | % rack position
      | len = norm(hp_wheel - hp_mt_rack);
      | x1 = asin(rad_pinion/len);
      | x2 = atan2(abs(hp_wheel(1) - hp_mt_rack(1)),hp_wheel(3) - hp_mt_rack(3));
      | pinion_incl = pi/2 - x2 + x1;
      | 
      | % Calcule pinion hardpoint 
      | hp_pinion = hp_mt_rack - [cos(pinion_incl) * rad_pinion, 0, sin(pinion_incl) * rad_pinion];
      | 
      | % Calculate location of universal joint
      | hp_ujoint = hp_wheel  - (hp_wheel - hp_pinion)/2;
      mask TypeOptions hp_wheel:
      | Ref to Wheel/Transform
      | HP Wheel/TranslationCartesianOffset
      mask TypeOptions hp_mt_rack:
      | Ref to Rack/Transform
      | HP Rack/TranslationCartesianOffset
      mask TypeOptions hp_out_rack: Rack/hp_out
      mask TypeOptions rack_mass: Rack/rack_mass
      mask TypeOptions whl2steer_filter: Physical Signal/InputFilterTimeConstant
      mask TypeOptions clr_rack: Rack/clr_rack
      mask TypeOptions opc_rack: Rack/opc_rack
      mask TypeOptions radius_rack: Rack/radius_rack
      mask TypeOptions clr_shaft:
      | Shaft
      | Steering/Shaft/GraphicDiffuseColor | Shaft
      | Lower/Shaft/GraphicDiffuseColor | Shaft
      | Intermediate/Shaft/GraphicDiffuseColor
      mask TypeOptions opc_shaft:
      | Shaft
      | Steering/Shaft/GraphicOpacity | Shaft
      | Lower/Shaft/GraphicOpacity | Shaft
      | Intermediate/Shaft/GraphicOpacity
      mask TypeOptions size_shaft:
      | Shaft
      | Steering/Shaft/CylinderRadius | Shaft
      | Lower/Shaft/CylinderRadius | Shaft
      | Intermediate/Shaft/CylinderRadius
      mask TypeOptions clr_pinion: Pinion/Pinion/GraphicDiffuseColor
      mask TypeOptions opc_pinion: Pinion/Pinion/GraphicOpacity
      mask TypeOptions len_pinion: Pinion/Pinion/CylinderLength
      mask TypeOptions clr_connhp:
      | Ref to Rack/Vis
      | Rack
      | Housing/GraphicDiffuseColor | HPs/HP Lower Col/GraphicDiffuseColor | HPs/HP Pinion/GraphicDiffuseColor | HPs/HP Upper Col/GraphicDiffuseColor
      mask TypeOptions opc_connhp:
      | Ref to Rack/Vis
      | Rack
      | Housing/GraphicOpacity | HPs/HP Lower Col/GraphicOpacity | HPs/HP Pinion/GraphicOpacity | HPs/HP Upper Col/GraphicOpacity
      mask TypeOptions size_connhp:
      | Ref to Rack/Vis
      | Rack
      | Housing/SphereRadius | HPs/HP Lower Col/SphereRadius | HPs/HP Pinion/SphereRadius | HPs/HP Upper Col/SphereRadius
      mask TypeOptions clr_wheel: Wheel/clr_wheel
      mask TypeOptions opc_wheel: Wheel/opc_wheel
      mask DialogControl cont_steer Prompt: Steer
      mask DialogControl grp_strparts Prompt: Parts
      mask DialogControl text_strparts_len Prompt: Length/Radius (m)
      mask DialogControl text_strparts_mass Prompt: Mass (kg)
      mask DialogControl text_strparts_wheel Prompt: Wheel
      mask DialogControl text_strparts_wheel_m Prompt: <CAD file>
      mask DialogControl text_strparts_sha_u Prompt: Upper Shaft
      mask DialogControl text_strparts_sha_i Prompt: Lower Shaft
      mask DialogControl text_strparts_sha_i_len Prompt: <length upper, lower>
      mask DialogControl text_strparts_pinion Prompt: Pinion
      mask DialogControl text_strparts_rack Prompt: Rack
      mask DialogControl text_strparts_rack_len Prompt: <HP Rod Inboard>
      mask DialogControl grp_steering Prompt: Steering Input
      mask DialogControl cont_vis_steer Prompt: Visualization
      mask DialogControl text_steer_vis_clr Prompt: Color [RGB]
      mask DialogControl text_steer_vis_opc Prompt: Opac. (0-1)
      mask DialogControl text_steer_vis_size Prompt: Size (m)
      mask DialogControl text_steer_vis_rack Prompt: Rack
      mask DialogControl text_steer_vis_shafts Prompt: Shafts
      mask DialogControl text_steer_vis_pinion Prompt: Pinion
      mask DialogControl text_steer_vis_connhp Prompt: Connections, HP
      mask DialogControl text_steer_vis_wheel Prompt: Wheel
      mask DialogControl text_steer_size_wheel Prompt: <CAD File>
      mask DialogControl cont_driver_human Prompt: Driver Human
  " rodL" : PMIOPort  Side=Right
  " ref" : PMIOPort  Port=2  Side=Right
  " rodR" : PMIOPort  Port=3  Side=Right
  " meas" : Outport  VectorParamsAs1DForOutWhenUnconnected=off

== system Linkage/Susp/Linkage/Wheel Meas Left ==
  note: For Steering Axis Inclination Estimation
  Bus Creator : BusCreator  Inputs=4
  Calculate Camber : Subsystem
  Calculate Camber Z Axis : Subsystem
  Calculate Toe : Subsystem
  Calculate Toe X Axis : Subsystem
  PS-Simulink Converter1 : nesl_utility/PS-Simulink Converter  PhysicalDomain=network_engine_domain  SubClassName=ps_output  LeftPortType=input  RightPortType=output  PseudoPeriodic=off  Frequencies=[]  VectorFormat=1-D array  Unit=1  AffineConversion=off
  Select x axis : Selector  NumberOfDimensions=2  InputPortWidth=2  IndexOptions=Index vector (dialog),Index vector (dialog)  Indices=[1 2 3],1  OutputSizes=1,1
  Select z axis : Selector  NumberOfDimensions=2  InputPortWidth=2  IndexOptions=Index vector (dialog),Index vector (dialog)  Indices=[1 2 3],3  OutputSizes=1,1
  Sign LR aCamber : Gain  Gain=180/pi*rhs_tc
  Sign LR aCamberX : Gain  Gain=180/pi*rhs_tc
  Sign LR aToe : Gain  Gain=180/pi*rhs_tc
  Sign LR aToeX : Gain  Gain=180/pi*rhs_tc
  Transform Sensor : sm_lib/Frames and Transforms/Transform Sensor  MeasurementFrame=Base  RotationSequence=XYX  SenseAngle=off  SenseAxis=off  SenseQ=off  SenseR=on  SenseRotationSequence=off  SenseOmegaX=off  SenseOmegaY=off  SenseOmegaZ=off  SenseOmega=off  SenseQDot=off  SenseRDot=off  SenseRotationSequenceDot=off  SenseAlphaX=off  SenseAlphaY=off  SenseAlphaZ=off  SenseAlpha=off  SenseQDDot=off  SenseRDDot=off  SenseX=off  SenseY=off  SenseZ=off  SenseXYZ=off  SenseRad=off  SenseAzim=off  SenseDist=off  SenseInc=off  SenseXDot=off  SenseYDot=off  SenseZDot=off  SenseXYZDot=off  SenseRadDot=off  SenseAzimDot=off  SenseDistDot=off  SenseIncDot=off  SenseXDDot=off  SenseYDDot=off  SenseZDDot=off  SenseXYZDDot=off  SenseRadDDot=off  SenseAzimDDot=off  SenseDistDDot=off  SenseIncDDot=off
  Ref : PMIOPort  Side=Left
  Whl Ctr : PMIOPort  Port=2  Side=Left
  meas : Outport  VectorParamsAs1DForOutWhenUnconnected=off
  wires:
  Calculate Toe/1(Toe) -> Sign LR aToe/1
  Calculate Camber/1(Camber) -> Sign LR aCamber/1
  Select z axis/1 -> Calculate Toe/1(uvec spin axis), Calculate Camber/1(uvec spin axis)  "uvec spin axis"
  PS-Simulink Converter1/1 -> Select z axis/1, Select x axis/1
  Sign LR aCamber/1 -> Bus Creator/2  "aCamber"
  Sign LR aToe/1 -> Bus Creator/1  "aToe"
  Bus Creator/1 -> meas/1  "Whl"
  Sign LR aToeX/1 -> Bus Creator/3  "aToeX"
  Select x axis/1 -> Calculate Camber Z Axis/1(uvec spin axis), Calculate Toe X Axis/1(uvec spin axis)
  Sign LR aCamberX/1 -> Bus Creator/4  "aCamberX"
  Calculate Camber Z Axis/1(Camber) -> Sign LR aCamberX/1
  Calculate Toe X Axis/1(Toe) -> Sign LR aToeX/1
  connections:
  PS-Simulink Converter1/LConn1 -- Transform Sensor/RConn2
  Transform Sensor/RConn1 -- Whl Ctr/RConn1
  Transform Sensor/LConn1 -- Ref/RConn1

== system Linkage/Susp/Linkage/Wheel Meas Right ==
  note: For Steering Axis Inclination Estimation
  Bus Creator : BusCreator  Inputs=4
  Calculate Camber : Subsystem
  Calculate Camber Z Axis : Subsystem
  Calculate Toe : Subsystem
  Calculate Toe X Axis : Subsystem
  PS-Simulink Converter1 : nesl_utility/PS-Simulink Converter  PhysicalDomain=network_engine_domain  SubClassName=ps_output  LeftPortType=input  RightPortType=output  PseudoPeriodic=off  Frequencies=[]  VectorFormat=1-D array  Unit=1  AffineConversion=off
  Select x axis : Selector  NumberOfDimensions=2  InputPortWidth=2  IndexOptions=Index vector (dialog),Index vector (dialog)  Indices=[1 2 3],1  OutputSizes=1,1
  Select z axis : Selector  NumberOfDimensions=2  InputPortWidth=2  IndexOptions=Index vector (dialog),Index vector (dialog)  Indices=[1 2 3],3  OutputSizes=1,1
  Sign LR aCamber : Gain  Gain=180/pi*rhs_tc
  Sign LR aCamberX : Gain  Gain=180/pi*rhs_tc
  Sign LR aToe : Gain  Gain=180/pi*rhs_tc
  Sign LR aToeX : Gain  Gain=180/pi*rhs_tc
  Transform Sensor : sm_lib/Frames and Transforms/Transform Sensor  MeasurementFrame=Base  RotationSequence=XYX  SenseAngle=off  SenseAxis=off  SenseQ=off  SenseR=on  SenseRotationSequence=off  SenseOmegaX=off  SenseOmegaY=off  SenseOmegaZ=off  SenseOmega=off  SenseQDot=off  SenseRDot=off  SenseRotationSequenceDot=off  SenseAlphaX=off  SenseAlphaY=off  SenseAlphaZ=off  SenseAlpha=off  SenseQDDot=off  SenseRDDot=off  SenseX=off  SenseY=off  SenseZ=off  SenseXYZ=off  SenseRad=off  SenseAzim=off  SenseDist=off  SenseInc=off  SenseXDot=off  SenseYDot=off  SenseZDot=off  SenseXYZDot=off  SenseRadDot=off  SenseAzimDot=off  SenseDistDot=off  SenseIncDot=off  SenseXDDot=off  SenseYDDot=off  SenseZDDot=off  SenseXYZDDot=off  SenseRadDDot=off  SenseAzimDDot=off  SenseDistDDot=off  SenseIncDDot=off
  Ref : PMIOPort  Side=Left
  Whl Ctr : PMIOPort  Port=2  Side=Left
  meas : Outport  VectorParamsAs1DForOutWhenUnconnected=off
  wires:
  Calculate Toe/1(Toe) -> Sign LR aToe/1
  Calculate Camber/1(Camber) -> Sign LR aCamber/1
  Select z axis/1 -> Calculate Toe/1(uvec spin axis), Calculate Camber/1(uvec spin axis)  "uvec spin axis"
  PS-Simulink Converter1/1 -> Select z axis/1, Select x axis/1
  Sign LR aCamber/1 -> Bus Creator/2  "aCamber"
  Sign LR aToe/1 -> Bus Creator/1  "aToe"
  Bus Creator/1 -> meas/1  "Whl"
  Sign LR aToeX/1 -> Bus Creator/3  "aToeX"
  Select x axis/1 -> Calculate Camber Z Axis/1(uvec spin axis), Calculate Toe X Axis/1(uvec spin axis)
  Sign LR aCamberX/1 -> Bus Creator/4  "aCamberX"
  Calculate Camber Z Axis/1(Camber) -> Sign LR aCamberX/1
  Calculate Toe X Axis/1(Toe) -> Sign LR aToeX/1
  connections:
  PS-Simulink Converter1/LConn1 -- Transform Sensor/RConn2
  Transform Sensor/RConn1 -- Whl Ctr/RConn1
  Transform Sensor/LConn1 -- Ref/RConn1
